simulink model "f1_lap_dynamics_model"  (R2026a)
settings: Solver=FixedStepDiscrete  StartTime=0  StopTime=56  FixedStep=1
undefined symbols (not defined in the file): base_lap_time_seconds, fuel_gain_per_lap_seconds, initial_fuel_penalty_seconds, initial_tyre_age_laps, pace_offset_seconds, pit_loss_seconds, tyre_degradation_seconds_per_lap
settings Model: Creator=kyle_  LastModifiedBy=kyle_

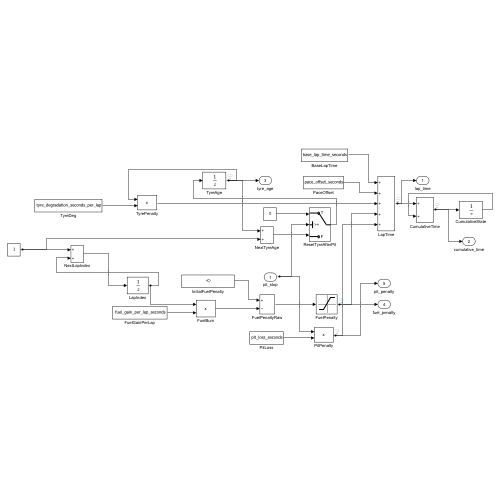
[thumbnail: Simulink's stored preview of the top-level diagram]
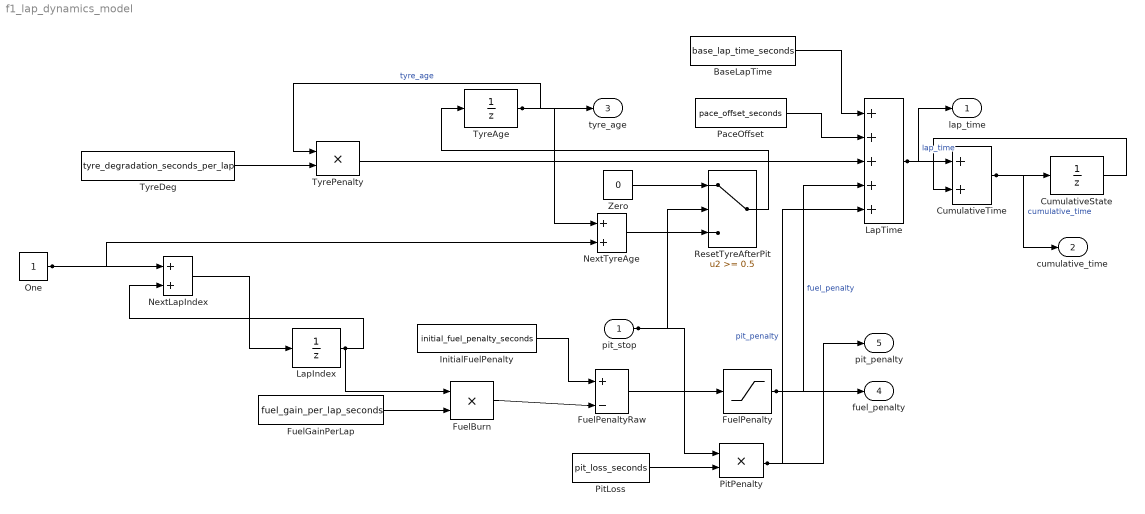
== system f1_lap_dynamics_model ==
  pit_stop : Inport
  BaseLapTime : Constant  Value=base_lap_time_seconds  SampleTime=1
  CumulativeState : UnitDelay
  CumulativeTime : Sum
  FuelBurn : Product
  FuelGainPerLap : Constant  Value=fuel_gain_per_lap_seconds  SampleTime=1
  FuelPenalty : Saturate  UpperLimit=inf  LowerLimit=0
  FuelPenaltyRaw : Sum  Inputs=+-
  InitialFuelPenalty : Constant  Value=initial_fuel_penalty_seconds  SampleTime=1
  LapIndex : UnitDelay
  LapTime : Sum  Inputs=+++++
  NextLapIndex : Sum
  NextTyreAge : Sum
  One : Constant  SampleTime=1
  PaceOffset : Constant  Value=pace_offset_seconds  SampleTime=1
  PitLoss : Constant  Value=pit_loss_seconds  SampleTime=1
  PitPenalty : Product
  ResetTyreAfterPit : Switch  Threshold=0.5  SaturateOnIntegerOverflow=off  InputSameDT=off
  TyreAge : UnitDelay  InitialCondition=initial_tyre_age_laps
  TyreDeg : Constant  Value=tyre_degradation_seconds_per_lap  SampleTime=1
  TyrePenalty : Product
  Zero : Constant  Value=0  SampleTime=1
  lap_time : Outport
  cumulative_time : Outport  Port=2
  tyre_age : Outport  Port=3
  fuel_penalty : Outport  Port=4
  pit_penalty : Outport  Port=5
  wires:
  PaceOffset/1 -> LapTime/2
  PitLoss/1 -> PitPenalty/2
  InitialFuelPenalty/1 -> FuelPenaltyRaw/1
  BaseLapTime/1 -> LapTime/1
  One/1 -> NextTyreAge/2, NextLapIndex/1
  TyreDeg/1 -> TyrePenalty/2
  FuelGainPerLap/1 -> FuelBurn/2
  FuelBurn/1 -> FuelPenaltyRaw/2
  NextLapIndex/1 -> LapIndex/1
  ResetTyreAfterPit/1 -> TyreAge/1
  TyrePenalty/1 -> LapTime/3
  LapIndex/1 -> NextLapIndex/2, FuelBurn/1
  NextTyreAge/1 -> ResetTyreAfterPit/3
  TyreAge/1 -> TyrePenalty/1, NextTyreAge/1, tyre_age/1  "tyre_age"
  Zero/1 -> ResetTyreAfterPit/1
  pit_stop/1 -> ResetTyreAfterPit/2, PitPenalty/1
  FuelPenaltyRaw/1 -> FuelPenalty/1
  FuelPenalty/1 -> LapTime/4, fuel_penalty/1  "fuel_penalty"
  LapTime/1 -> CumulativeTime/1, lap_time/1  "lap_time"
  PitPenalty/1 -> LapTime/5, pit_penalty/1  "pit_penalty"
  CumulativeState/1 -> CumulativeTime/2
  CumulativeTime/1 -> cumulative_time/1, CumulativeState/1  "cumulative_time"
